simulink model "networked"  (Simulink 7.4)
settings: Solver=ode45  StartTime=0.0  StopTime=2  RelTol=1e-3
libraries: truetime x5
settings Model: Creator=anton  LastModifiedBy=etu-adm  ExtModeAutoUpdateStatusClock=off
settings OptimizationCC: BooleanDataType=off
settings DebuggingCC: SaveWithParameterizedLinksMsg=none  SignalResolutionControl=TryResolveAllWithWarning  SolverPrmCheckMsg=none  MultiTaskDSMMsg=warning  MultiTaskCondExecSysMsg=none  StrictBusMsg=None
settings HardwareCC: TargetUnknown=on
settings RTWCC: IncludeERTFirstTime=on

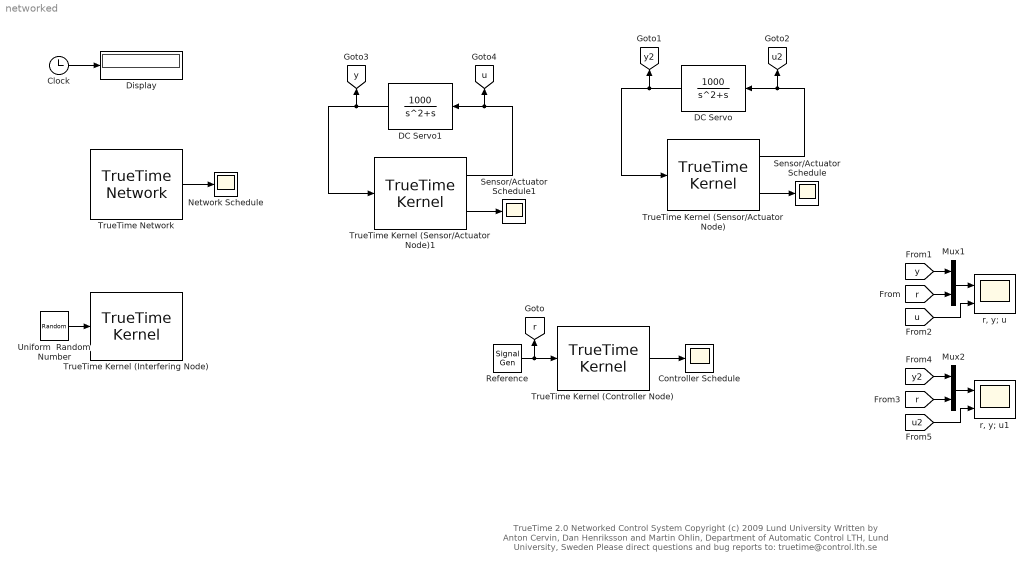
== system networked ==
  note: TrueTime 2.0  Networked Control System
      | Copyright (c) 2009 Lund University
      | Written by Anton Cervin, Dan Henriksson and Martin Ohlin,
      | Department of Automatic Control LTH, Lund University, Sweden
      | Please direct questions and bug reports to:  truetime@control.lth.se
  Clock : Clock
      settings: Decimation=10
  Controller Schedule : Scope
      settings: TimeRange=2  YMin=0.5  YMax=4  SaveName=nschedule
  DC Servo : TransferFcn  Numerator=[1000]  Denominator=[1 1 0]
  DC Servo1 : TransferFcn  Numerator=[1000]  Denominator=[1 1 0]
  Display : Display
  Mux1 : Mux  Inputs=2
  Mux2 : Mux  Inputs=2
  Network Schedule : Scope
      settings: TimeRange=2  YMin=1  YMax=3.5  SaveName=nschedule1
  Reference : SignalGenerator  WaveForm=square
  Sensor/Actuator Schedule : Scope
      settings: TimeRange=2  YMin=0.5  YMax=4  SaveName=nschedule3
  Sensor/Actuator Schedule1 : Scope
      settings: TimeRange=2  YMin=0.5  YMax=4  SaveName=nschedule2
  TrueTime Kernel (Controller Node) : truetime/TrueTime Kernel  SystemSampleTime=-1  sfun=controller_init  args=0.0  ninputsoutputs=[1 0]  ntriggers=0  trigtype=rising  nwnodenbr=3  clockoffsetdrift=[0 0]  schedoutput=on  battery=off  poweroutput=off  label=1: 3
  TrueTime Kernel (Interfering Node) : truetime/TrueTime Kernel  SystemSampleTime=-1  sfun=interference_init  args=0.0  ninputsoutputs=[1 0]  ntriggers=0  trigtype=rising  nwnodenbr=1  clockoffsetdrift=[0 0]  schedoutput=off  battery=off  poweroutput=off  label=1: 1
  TrueTime Kernel (Sensor/Actuator Node) : truetime/TrueTime Kernel  SystemSampleTime=-1  sfun=sensor_actuator_init2  args=[]  ninputsoutputs=[1 1]  ntriggers=0  trigtype=rising  nwnodenbr=4  clockoffsetdrift=[0 0]  schedoutput=on  battery=off  poweroutput=off  label=1: 2
  TrueTime Kernel (Sensor/Actuator Node)1 : truetime/TrueTime Kernel  SystemSampleTime=-1  sfun=sensor_actuator_init  args=[]  ninputsoutputs=[1 1]  ntriggers=0  trigtype=rising  nwnodenbr=2  clockoffsetdrift=[0 0]  schedoutput=on  battery=off  poweroutput=off  label=1: 2
  TrueTime Network : truetime/TrueTime Network  SystemSampleTime=-1  nwtype=CSMA/CD (Ethernet)  nwnbr=1  nnodes=4  rate=80000  minsize=80  lossprob=0  seed=0  bandwidths=[0.5 0.25 0.25]  slotsize=80  schedule=[1 2 1 3]  memsize=80000  buftype=Common buffer  overflow=Retransmit  dynSchedule=[]  miniSlotSize=40  NIT=0  QSortMode=FIFO  sync=0  irtSchedule=0  nrtLength=0  nodeGraph=0  scheduleoutput=on
  Uniform  Random Number : UniformRandomNumber  Minimum=0  SampleTime=0.001
  "r, y; u" : Scope  NumInputPorts=2
      settings: TimeRange=2  YMin=-2~-3  YMax=2~3  SaveName=y
  "r, y; u1" : Scope  NumInputPorts=2
      settings: TimeRange=2  YMin=-2~-3  YMax=2~3  SaveName=y1
  tag scope: r=global, u2=global, u=global, y2=global, y=global
  wires:
  TrueTime Network/1 -> Network Schedule/1
  Mux1/1 -> "r, y; u"/1
  Clock/1 -> Display/1
  Reference/1 -> TrueTime Kernel (Controller Node)/1, [r]
  TrueTime Kernel (Controller Node)/1 -> Controller Schedule/1
  [r] -> Mux1/2
  [y] -> Mux1/1
  [u] -> "r, y; u"/2
  Uniform  Random Number/1 -> TrueTime Kernel (Interfering Node)/1
  TrueTime Kernel (Sensor/Actuator Node)/2 -> Sensor/Actuator Schedule/1
  DC Servo/1 -> TrueTime Kernel (Sensor/Actuator Node)/1, [y2]
  TrueTime Kernel (Sensor/Actuator Node)/1 -> DC Servo/1, [u2]
  TrueTime Kernel (Sensor/Actuator Node)1/2 -> Sensor/Actuator Schedule1/1
  DC Servo1/1 -> [y], TrueTime Kernel (Sensor/Actuator Node)1/1
  TrueTime Kernel (Sensor/Actuator Node)1/1 -> [u], DC Servo1/1
  Mux2/1 -> "r, y; u1"/1
  [r] -> Mux2/2
  [y2] -> Mux2/1
  [u2] -> "r, y; u1"/2
